simulink model "NonlinearDesignModel"  (R2025a)
settings: Solver=VariableStepAuto  StartTime=0.0  StopTime=10.0  RelTol=1e-3
values from neighbouring files (symbols this model uses):
  K_pd = -(lambda_1 + lambda_2) / K_1    (= 7.72018348624)    [init_heli_part3.m]    (also in simDesignModel.m = -(lambda_1 + lambda_2) / K_1)
  K_pp = (lambda_1 * lambda_2) / K_1    (= 7.72018348624)    [init_heli_part3.m]    (also in simDesignModel.m = (lambda_1 * lambda_2) / K_1)
  L_1 = l_p * K_f    (= 0.022849197861)    [init_heli_3_10.m]    (also in init_heli_part3.m)
  L_4 = l_h * K_f    (= 0.0861741176471)    [init_heli_3_10.m]
undefined symbols (not defined in the file or in its folder): L_2, L_3
settings Model: Creator=ole  LastModifiedBy=ole

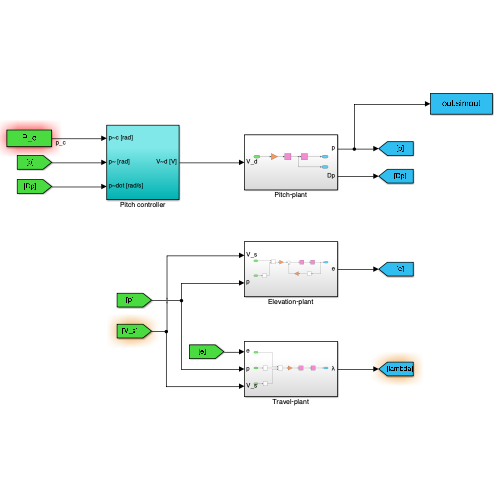
[thumbnail: Simulink's stored preview of the top-level diagram]
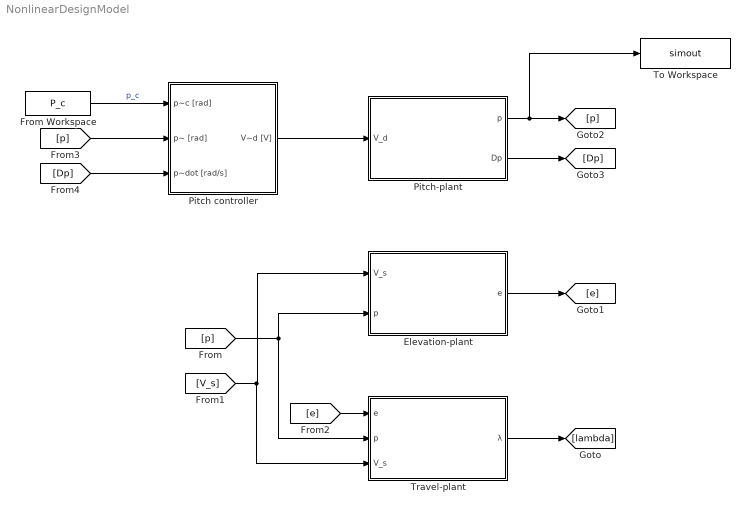
== system NonlinearDesignModel ==
  Elevation-plant : Subsystem
  From Workspace : FromWorkspace  VariableName=P_c
  Pitch controller : Subsystem
  Pitch-plant : Subsystem
  To Workspace : ToWorkspace  VariableName=simout  SaveFormat=Timeseries  SampleTime=-1
  Travel-plant : Subsystem
  wires:
  Pitch controller/1(V~d [V]) -> Pitch-plant/1(V_d)
  Pitch-plant/1(p) -> To Workspace/1, [p]
  Pitch-plant/2(Dp) -> [Dp]
  From Workspace/1 -> Pitch controller/1(p~c [rad])  "p_c"
  Elevation-plant/1(e) -> [e]
  Travel-plant/1(λ) -> [lambda]
  [V_s] -> Travel-plant/3(V_s), Elevation-plant/1(V_s)
  [e] -> Travel-plant/1(e)
  [p] -> Elevation-plant/2(p), Travel-plant/2(p)
  [p] -> Pitch controller/2(p~ [rad])
  [Dp] -> Pitch controller/3(p~dot [rad/s])

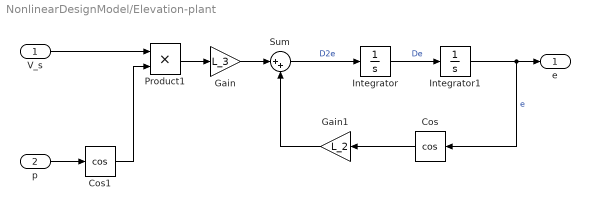
== system NonlinearDesignModel/Elevation-plant ==
  V_s : Inport
  p : Inport  Port=2
  Cos : Trigonometry  Operator=cos
  Cos1 : Trigonometry  Operator=cos
  Gain : Gain  Gain=L_3
  Gain1 : Gain  Gain=L_2
  Integrator : Integrator
  Integrator1 : Integrator
  Product1 : Product
  Sum : Sum  Inputs=|++
  e : Outport
  wires:
  Integrator1/1 -> Cos/1, e/1  "e"
  V_s/1 -> Product1/1
  Integrator/1 -> Integrator1/1  "De"
  Sum/1 -> Integrator/1  "D2e"
  Gain1/1 -> Sum/2
  Cos/1 -> Gain1/1
  p/1 -> Cos1/1
  Cos1/1 -> Product1/2
  Product1/1 -> Gain/1
  Gain/1 -> Sum/1

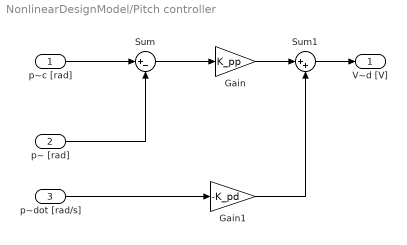
== system NonlinearDesignModel/Pitch controller ==
  p~c [rad] : Inport
  p~ [rad] : Inport  Port=2
  p~dot [rad/s] : Inport  Port=3
  Gain : Gain  Gain=K_pp
  Gain1 : Gain  Gain=-K_pd
  Sum : Sum  Inputs=|+-
  Sum1 : Sum  Inputs=|++
  V~d [V] : Outport  InitialOutput=0
  wires:
  Sum/1 -> Gain/1
  p~ [rad]/1 -> Sum/2
  p~dot [rad/s]/1 -> Gain1/1
  Gain/1 -> Sum1/1
  Gain1/1 -> Sum1/2
  p~c [rad]/1 -> Sum/1
  Sum1/1 -> V~d [V]/1

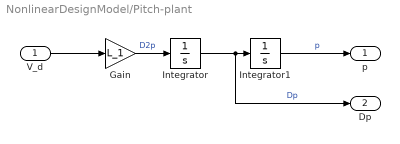
== system NonlinearDesignModel/Pitch-plant ==
  V_d : Inport
  Gain : Gain  Gain=L_1
  Integrator : Integrator
  Integrator1 : Integrator
  p : Outport
  Dp : Outport  Port=2
  wires:
  Integrator1/1 -> p/1  "p"
  V_d/1 -> Gain/1
  Integrator/1 -> Dp/1, Integrator1/1  "Dp"
  Gain/1 -> Integrator/1  "D2p"

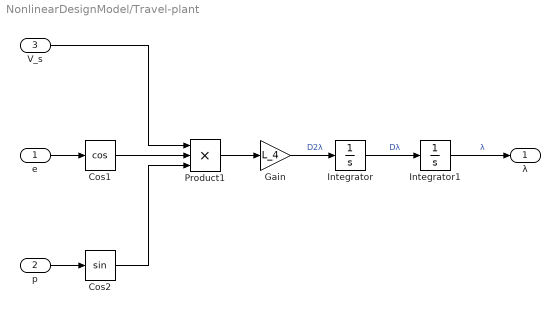
== system NonlinearDesignModel/Travel-plant ==
  e : Inport
  p : Inport  Port=2
  V_s : Inport  Port=3
  Cos1 : Trigonometry  Operator=cos
  Cos2 : Trigonometry
  Gain : Gain  Gain=L_4
  Integrator : Integrator
  Integrator1 : Integrator
  Product1 : Product  Inputs=3
  λ : Outport
  wires:
  Integrator1/1 -> λ/1  "λ"
  e/1 -> Cos1/1
  Integrator/1 -> Integrator1/1  "Dλ"
  Gain/1 -> Integrator/1  "D2λ"
  p/1 -> Cos2/1
  Cos2/1 -> Product1/3
  Product1/1 -> Gain/1
  Cos1/1 -> Product1/2
  V_s/1 -> Product1/1
